simulink model "CPR_Controller"  (R2024b)
settings: Solver=VariableStepAuto  StartTime=0.0  StopTime=3  MaxStep=0.00001  RelTol=1e-6
values from neighbouring files (symbols this model uses):
  k = 1    [nyqlog.m]
  R = R/spiralfactor    (= 6.66666666667e-06)    [nyqlog.m]
undefined symbols (not defined in the file or in its folder): b, c, denom_discrete, dspblkCoreblockFVToolHelper, gcbh, gear_ratio, J, K_i, K_p, K_torque, m, num_discrete, plant_denom, plant_num, T
libraries: dspsigops x1, simulink x1
settings Model: Creator=jonat  LastModifiedBy=danie

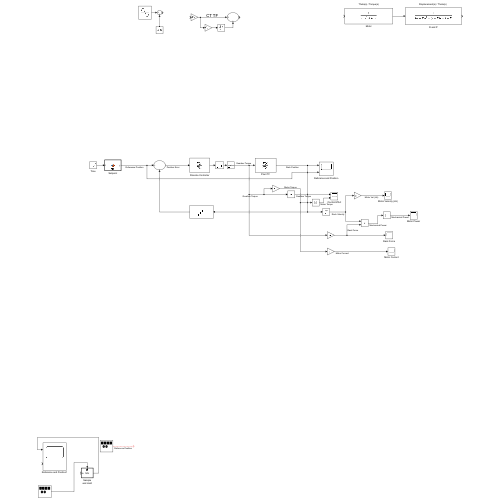
[thumbnail: Simulink's stored preview of the top-level diagram]
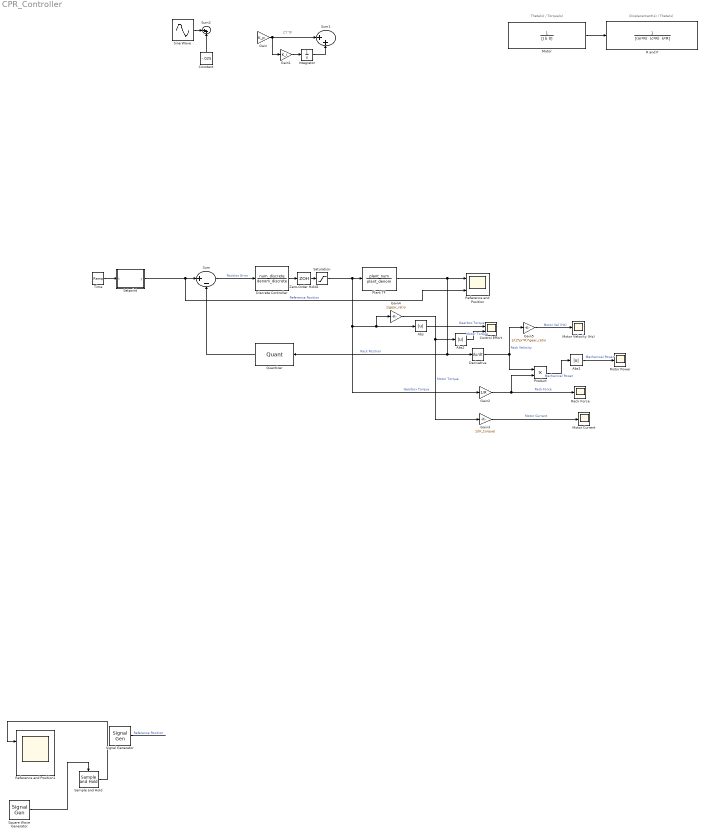
== system CPR_Controller ==
  note: CT TF
  note: Displacement(s) / Theta(s)
  note: Theta(s) / Torque(s)
  Abs : Abs  SaturateOnIntegerOverflow=off
  Abs1 : Abs  SaturateOnIntegerOverflow=off
  Abs2 : Abs  SaturateOnIntegerOverflow=off
  Constant : Constant  Value=-.025
  Control Effort : Scope  NumInputPorts=2
  Derivative : Derivative
  Discrete Controller : DiscreteTransferFcn  LoadFcn=dspblkCoreblockFVToolHelper(gcbh,'load');  Numerator=num_discrete  Denominator=denom_discrete
      settings: CopyFcn=dspblkCoreblockFVToolHelper(gcbh,'copy');  DeleteFcn=dspblkCoreblockFVToolHelper(gcbh,'close');  ModelCloseFcn=dspblkCoreblockFVToolHelper(gcbh,'close');  PreSaveFcn=dspblkCoreblockFVToolHelper(gcbh,'presave');  PostSaveFcn=dspblkCoreblockFVToolHelper(gcbh,'postsave');  CloseFcn=dspblkCoreblockFVToolHelper(gcbh,'close');
  Gain : Gain  Gain=K_p
  Gain1 : Gain  Gain=K_i
  Gain2 : Gain  Gain=1/R
  Gain3 : Gain  Gain=1/(K_torque)
  Gain4 : Gain  Gain=1/gear_ratio
  Gain5 : Gain  Gain=1/(2*pi*R)*gear_ratio
  Integrator : Integrator  LimitOutput=on  UpperSaturationLimit=5  LowerSaturationLimit=-5
  Motor : TransferFcn  Denominator=[J b 0]
  Motor Current : Scope
  Motor Power : Scope
  Motor Velocity (Hz) : Scope
  Plant TF : TransferFcn  Numerator=plant_num  Denominator=plant_denom
  Product : Product
  Quantizer : Quantizer  QuantizationInterval=0.0005
  R and P : TransferFcn  Denominator="[(m*R)  (c*R)  k*R]"
  Rack Force : Scope
  Reference and Position : Scope  NumInputPorts=2
  Reference and Position1 : Scope  NumInputPorts=2
  Sample and Hold : dspsigops/Sample and Hold  trig=Rising edge  initCond=0  latchinput=off
  Saturation : Saturate  UpperLimit=5  LowerLimit=-5
  Setpoint : MATLAB Function  TreatAsAtomicUnit=on
  Signal Generator : SignalGenerator  Amplitude=.05/2  Frequency=2
  Sine Wave : Sin  Amplitude=.05/2  Frequency=2*pi*2  Phase=pi/2  SampleTime=0  VectorParams1D=off
  Square Wave Generator : SignalGenerator  WaveForm=square  Frequency=1/T
  Sum : Sum  Inputs=|+-
  Sum1 : Sum  Inputs=|++
  Sum2 : Sum  Inputs=|++
  Time : simulink/Sources/Ramp  slope=1  start=0  InitialOutput=0
  Zero-Order Hold2 : ZeroOrderHold  SampleTime=T
  wires:
  Plant TF/1 -> Reference and Position/1, Quantizer/1, Derivative/1  "Rack Position"
  Motor/1 -> R and P/1
  Square Wave Generator/1 -> Sample and Hold/Trigger
  Sample and Hold/1 -> Reference and Position1/1
  Gain1/1 -> Integrator/1
  Gain/1 -> Gain1/1, Sum1/1
  Integrator/1 -> Sum1/2
  Saturation/1 -> Gain4/1, Abs/1, Gain2/1, Plant TF/1  "Gearbox Torque"
  Derivative/1 -> Gain5/1, Product/1  "Rack Velocity"
  Gain2/1 -> Rack Force/1, Product/2  "Rack Force"
  Product/1 -> Abs1/1  "Mechanical Power"
  Quantizer/1 -> Sum/2
  Sum/1 -> Discrete Controller/1  "Position Error"
  Discrete Controller/1 -> Zero-Order Hold2/1
  Signal Generator/1 -> ?  "Reference Position"
  Zero-Order Hold2/1 -> Saturation/1
  Gain3/1 -> Motor Current/1  "Motor Current"
  Sine Wave/1 -> Sum2/1
  Constant/1 -> Sum2/2
  Gain4/1 -> Gain3/1, Abs2/1  "Motor Torque"
  Abs1/1 -> Motor Power/1  "Mechanical Power"
  Gain5/1 -> Motor Velocity (Hz)/1  "Motor Vel (Hz)"
  Abs/1 -> Control Effort/1  "Gearbox Torque"
  Abs2/1 -> Control Effort/2  "Motor Torque"
  Time/1 -> Setpoint/1(t)
  Setpoint/1(y) -> Reference and Position/2, Sum/1  "Reference Position"

== matlab function CPR_Controller/Setpoint ==
  data: t input; y output
function y = fcn(t)
    time = mod(t, .56);
    
    if (time <= .12)
        y = 0;
    elseif (time <= .24)
        y = (-41.6666667*(time - .12))*1e-2;
    elseif (time <= .323)
        y = -5e-2;
    else
        y = (21.0965609*(time - .323) - 5)*1e-2;
    end
end
